simulink model "prova"  (Simulink 6.5)
settings: Solver=FixedStepDiscrete  StartTime=0.0  StopTime=10.0  FixedStep=0.001  RelTol=1e-3
libraries: dsPICdrivers x12
settings Model: Creator=Manu  LastModifiedBy=Manu  ProdHWDeviceType=16-bit Generic
settings OptimizationCC: OptimizeModelRefInitCode=on  LifeSpan=1
settings HardwareCC: ProdBitPerInt=16  ProdEndianess=LittleEndian  ProdWordSize=16  ProdHWDeviceType=16-bit Generic  TargetHWDeviceType=32-bit Generic
settings RTWCC: SystemTargetFile=dspic.tlc  TemplateMakefile=dspic_pic30_gcc.tmf  PostCodeGenCommand=dsPIC_Compile()  Description=Embedded Target for Microchip dsPIC (real-time)  ProcessScript=dspic_make_rtw_hook
settings CodeAppCC: IgnoreCustomStorageClasses=off
settings STFCustomTargetCC: TargetFcnLib=ansi_tfl_tmw.mat  GenFloatMathFcnCalls=ANSI_C  ModelReferenceCompliant=off  IncludeMdlTerminateFcn=off  CombineOutputUpdateFcns=on  SuppressErrorStatus=on  ERTCustomFileBanners=on  SupportContinuousTime=off  SupportNonInlinedSFcns=off  SystemTargetFile=dspic.tlc
settings ERTTargetCC: TargetFcnLib=ansi_tfl_tmw.mat  GenFloatMathFcnCalls=ANSI_C  ModelReferenceCompliant=off  IncludeMdlTerminateFcn=off  SuppressErrorStatus=on  InlinedParameterPlacement=NonHierarchical  ERTSrcFileBannerTemplate=dsPIC_code_template.cgt  ERTHdrFileBannerTemplate=dsPIC_code_template.cgt  ERTDataSrcFileTemplate=dsPIC_code_template.cgt  ERTDataHdrFileTemplate=dsPIC_code_template.cgt  ERTCustomFileTemplate=dsPIC_main.tlc
settings CustomProperty: DataType=string  Value=C:\PROGRA~1\MATLAB\R2006b\rtw\bin\win32\gmake

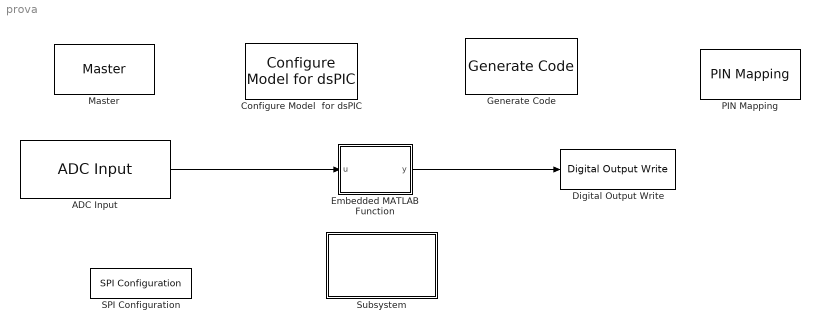
== system prova ==
  ADC Input : dsPICdrivers/Peripheral I//O/ADC Input  Tag=dsPIC_ADC  Priority=5  ADC_TYPE=10 bits  ADC_MODE=Continuous sampling & get last channel value  NbrSampleStep=1  VoltRefpopup="AVdd  -  AVss"  OutFormatBitspopup=0000 00dd dddd dddd : Integer  InterruptPriority=7  ANCHANNELS=[0]  MaxName=ANmax = 1024  Rin=1e2  ADCS=12  SAMC=1  Temperature=25  DMAChannel=0  SampleTime=-1  Status="OK  |  Tsmp=1.625e-007 |  T/Channel=2.113e-006 |  Tall=2.113e-006"
  Configure Model  for dsPIC : dsPICdrivers/Simulink Configuration/Configure Model  for dsPIC
  Digital Output Write : dsPICdrivers/Digital I//O/Digital Output Write  Tag=dsPIC_Digital_Output  Priority=5  PORT=B  Pin=[2]  Simultaneous=off  OrderingInOutPopup=None
  Embedded MATLAB Function : Stateflow chart
  Generate Code : dsPICdrivers/Simulink Configuration/Generate Code
  Master : dsPICdrivers/Master  Tag=dsPIC_MASTER  Priority=1  TimeStepType=Timer1  picType=33fj128GP802  fcy=40000000  Quartz_33f=20e6  PLLActive_33f=on  fcyDesired_33f=40000000  tmr1="[1  39999  0]"  tmr1Info="Time Step : 0.001  ;   Error : 0%  PR1=39999"  tmr2345="[0  0  0  0]"  tmr2345cfg=[-1 -1 -1 -1]  IOautoConf=on  typePort="[ 8   0   0   0   0   0   0   0   0   0   0   0   0   0   0   0   0   0  10   0   0   0   0   0   0   0  23  23  10   0   0   0   0   0   0   0   0   0   0   0   0   0   0   0   0   0   0   0   0   0   0   0   0   0   0   0   0   0   0   0   0   0   0   0   0   0   0   0   0   0   0   0   0   0   0   0   0   0   0   0   0   0   0   0   0   0   0   0   0   0   0   0   0   0   0   0   0   0   0   0   0   0   0   0   0   0   0   0   0   0   0   0 ]"  TRIS="[ 65535  58363  65535  65535  65535  65535  65535 ]"  ADPCFG=4112  MasterBusyPort=None  MasterOverloadPort=None  FOSC=Quartz (XT - HS)  ClockSwitchMonitor=Clock switching and monitor enabled  TempProtection_33f=TEMP_ON  FPBOR=<empty>  PWRT=32ms  MCLR=<empty>  PowerSave=off  OverrideFcy=off  NewFcy=1e6
  PIN Mapping : dsPICdrivers/Peripheral MAPPING/PIN Mapping  Tag=dsPIC_PIN_Mapping  in_INT1=Not tied (VSS)  in_INT2=Not tied (VSS)  in_T2CK=Not tied (VSS)  in_T3CK=Not tied (VSS)  in_T4CK=Not tied (VSS)  in_T5CK=Not tied (VSS)  in_IC1=Not tied (VSS)  in_IC2=Not tied (VSS)  in_IC7=Not tied (VSS)  in_IC8=Not tied (VSS)  out_OC1=Not changed  out_OC2=Not changed  out_OC3=Not changed  out_OC4=Not changed  in_OCFA=Not tied (VSS)  in_FLTA1=Not tied (VSS)  in_FLTA2=Not tied (VSS)  in_QEA1=Not tied (VSS)  in_QEB1=Not tied (VSS)  in_INDX1=Not tied (VSS)  out_UPDN1=Not changed  out_UPDN2=Not changed  in_QEA2=Not tied (VSS)  in_QEB2=Not tied (VSS)  in_INDX2=Not tied (VSS)  in_U1RX=Not tied (VSS)  out_U1TX=Not changed  in_U1CTS=Not tied (VSS)  out_U1RTS=Not changed  in_U2RX=Not tied (VSS)  out_U2TX=Not changed  in_U2CTS=Not tied (VSS)  out_U2RTS=Not changed  in_SDI1=Not tied (VSS)  out_SDO1=tied to RP10  in_SCK1=Not tied (VSS)  out_SCK1OUT=tied to RP11  in_SS1=Not tied (VSS)  out_SS1OUT=Not changed  in_SDI2=Not tied (VSS)  out_SDO2=Not changed  in_SCK2=Not tied (VSS)  out_SCK2OUT=Not changed  in_SS2=Not tied (VSS)  out_SS2OUT=Not changed  in_C1RX=Not tied (VSS)  out_C1TX=Not changed  out_C1OUT=Not changed  out_C2OUT=Not changed
  SPI Configuration : dsPICdrivers/SPI PORT/SPI Configuration  Tag=dsPIC_config_SPI  Priority=2  ConfigurationTime=At boot time (only once)  OrderingInOutPopup=None  SampleTime=-1  Frame_Enable=0  Frame_Sync=None  SPI=1  MODE=MASTER  USER_SCALER=8  StartEnable=Enable  SDO_EN=on  DATA_LENGTH=16 bits  SS_EN=off  SMP=Middle of bit  CKP=low  CKE=Idle to Active  Status="OK - Mode 3  -    Fsck= 5000000Hz"
  Subsystem : Subsystem  TreatAsAtomicUnit=on
  wires:
  Embedded MATLAB Function/1(y) -> Digital Output Write/1
  ADC Input/1 -> Embedded MATLAB Function/1(u)

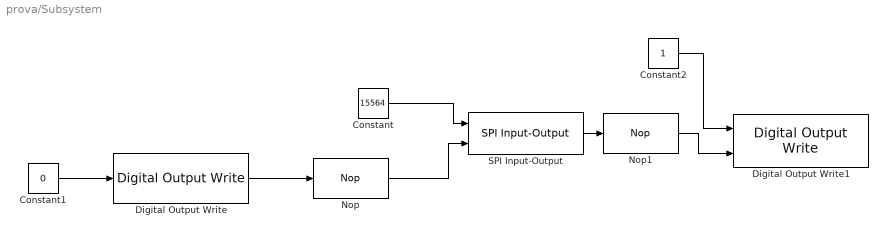
== system prova/Subsystem ==
  Constant : Constant  Value=15564  OutDataTypeMode=uint16  OutDataType=sfix(16)  ConRadixGroup=Use specified scaling  OutScaling=2^0  SampleTime=inf  FramePeriod=inf
  Constant1 : Constant  Value=0  OutDataTypeMode=boolean  OutDataType=sfix(16)  ConRadixGroup=Use specified scaling  OutScaling=2^0  SampleTime=inf  FramePeriod=inf
  Constant2 : Constant  Value=1  OutDataTypeMode=boolean  OutDataType=sfix(16)  ConRadixGroup=Use specified scaling  OutScaling=2^0  SampleTime=inf  FramePeriod=inf
  Digital Output Write : dsPICdrivers/Digital I//O/Digital Output Write  Tag=dsPIC_Digital_Output  Priority=5  PORT=B  Pin=[12]  Simultaneous=off  OrderingInOutPopup=Output
  Digital Output Write1 : dsPICdrivers/Digital I//O/Digital Output Write  Tag=dsPIC_Digital_Output  Priority=5  PORT=B  Pin=[12]  Simultaneous=off  OrderingInOutPopup=Input
  Nop : dsPICdrivers/OTHERS/Nop  Tag=dsPIC_Reset  NbrNop=5
  Nop1 : dsPICdrivers/OTHERS/Nop  Tag=dsPIC_Reset  NbrNop=5
  SPI Input-Output : dsPICdrivers/SPI PORT/SPI Input-Output  Tag=dsPIC_SPI  SPI=1  INPUT=off  RESET_INPUT=on  OUTPUT=on  SPECIAL_SPI=Always Enable  DATA_LENGTH=16 bits  WAIT_INPUTDATA=off  OrderingInOutPopup=Input & Output  SampleTime=-1
  wires:
  Constant/1 -> SPI Input-Output/1
  Digital Output Write/1 -> Nop/1
  Constant1/1 -> Digital Output Write/1
  Nop/1 -> SPI Input-Output/2
  SPI Input-Output/1 -> Nop1/1
  Nop1/1 -> Digital Output Write1/2
  Constant2/1 -> Digital Output Write1/1

== matlab function Embedded MATLAB Function ==
  data: u input inherited; y output boolean
function y = fcn(u)
% This block supports an embeddable subset of the MATLAB language.
% See the help menu for details. 
if (u <= 512)
    y = FALSE;
else
    y = TRUE;
end
